simulink model "ASM_Traffic_new"  (R2024a)
settings: Solver=ode1  StartTime=SIM.tstart.v  StopTime=SIM.tend.v  FixedStep=SIM.StepSize.v  RelTol=1e-3
PostLoadFcn:
  | if any(exist('dsrtsu_mdlpostloadfcn', 'file') ~= 0), dsrtsu_mdlpostloadfcn('Execute', bdroot); end
  | try, asm_mdl_postloadfcn(bdroot, 'UpdateModel', 3600); catch, disp(lasterr); end,
InitFcn:
  | , if any(exist('rtifpga_mdlclblib', 'file') ~= 0), rtifpga_mdlclblib('Init', bdroot); end,
  | , if any(exist('dsmpb_private', 'file') ~= 0), dsmpb_private('dsmpb_mdlclblib', 'Init', bdroot); end,
undefined symbols (not defined in the file): _to_, a0b2, ASM_BrakeHydraulics_DemoSystems, ASM_VehicleDynamics_DemoSystems, b98103fe8ad365046cd0, BrakeCircuit, CPT, Crankshaft, DiscIntNeverNeededParam, dsmsi, FinalDriveAssembly, MDL, ModeSignals, Pos_BrakePedal_Maneuver, rad, RefSignals, s_to_rpm, SIM, SoftECU, Suspension, Tire, Transmission
libraries: ASM_Traffic_lib x135, simulink x100, ASM_Utils_lib x77, ASM_VehicleDynamics_lib x70, ASM_Environment_lib x22, dsmpblib x20, dsmsilib x15, MDLD_Utils_lib x10, ASM_BrakeHydraulics_lib x3
(part 49 of 63)

== system ASM_Traffic_new/Environment/Sensors/UserInterface/DISP_Plant/Object_Sensor_2D/Object_Sensor_2D_VisualizationData ==
  TrafficBus : Inport
  Bus Selector9 : BusSelector  OutputSignals=Object_Sensor_2D.Sensor_1_Front,Object_Sensor_2D.Sensor_2_Front_Left,Object_Sensor_2D.Sensor_3_Left,Object_Sensor_2D.Sensor_4_Rear_Left,Object_Sensor_2D.Sensor_5_Front_Right,Object_Sensor_2D.Sensor_6_Right,Object_Sensor_2D.Sensor_7_Rear_Right
  Sensor_1_Front_Long : Subsystem
  Sensor_2_Front_Left : Subsystem
  Sensor_3_Left : Subsystem
  Sensor_4_Rear_Left : Subsystem
  Sensor_5_Front_Right : Subsystem
  Sensor_6_Right : Subsystem
  Sensor_7_Rear_Right : Subsystem
  wires:
  Bus Selector9/1 -> Sensor_1_Front_Long/1(Sensor)  "<Sensor_1_Front>"
  TrafficBus/1 -> Bus Selector9/1
  Bus Selector9/2 -> Sensor_2_Front_Left/1(Sensor)  "<Sensor_2_Front_Left>"
  Bus Selector9/3 -> Sensor_3_Left/1(Sensor)  "<Sensor_3_Left>"
  Bus Selector9/4 -> Sensor_4_Rear_Left/1(Sensor)  "<Sensor_4_Rear_Left>"
  Bus Selector9/5 -> Sensor_5_Front_Right/1(Sensor)  "<Sensor_5_Front_Right>"
  Bus Selector9/6 -> Sensor_6_Right/1(Sensor)  "<Sensor_6_Right>"
  Bus Selector9/7 -> Sensor_7_Rear_Right/1(Sensor)  "<Sensor_7_Rear_Right>"

== system ASM_Traffic_new/Environment/Sensors/UserInterface/DISP_Plant/Object_Sensor_2D/Object_Type[] ==
  In1 : Inport
  Out1 : Outport  VectorParamsAs1DForOutWhenUnconnected=off
  wires:
  In1/1 -> Out1/1

== system ASM_Traffic_new/Environment/Sensors/UserInterface/DISP_Plant/Object_Sensor_2D/Object_Type[]1 ==
  In1 : Inport
  Out1 : Outport  VectorParamsAs1DForOutWhenUnconnected=off
  wires:
  In1/1 -> Out1/1

== system ASM_Traffic_new/Environment/Sensors/UserInterface/DISP_Plant/Object_Sensor_2D/Object_Type[]2 ==
  In1 : Inport
  Out1 : Outport  VectorParamsAs1DForOutWhenUnconnected=off
  wires:
  In1/1 -> Out1/1

== system ASM_Traffic_new/Environment/Sensors/UserInterface/DISP_Plant/Object_Sensor_2D/Object_Type[]3 ==
  In1 : Inport
  Out1 : Outport  VectorParamsAs1DForOutWhenUnconnected=off
  wires:
  In1/1 -> Out1/1

== system ASM_Traffic_new/Environment/Sensors/UserInterface/DISP_Plant/Object_Sensor_2D/Object_Type[]4 ==
  In1 : Inport
  Out1 : Outport  VectorParamsAs1DForOutWhenUnconnected=off
  wires:
  In1/1 -> Out1/1

== system ASM_Traffic_new/Environment/Sensors/UserInterface/DISP_Plant/Object_Sensor_2D/Object_Type[]5 ==
  In1 : Inport
  Out1 : Outport  VectorParamsAs1DForOutWhenUnconnected=off
  wires:
  In1/1 -> Out1/1

== system ASM_Traffic_new/Environment/Sensors/UserInterface/DISP_Plant/Object_Sensor_2D/Object_Type[]6 ==
  In1 : Inport
  Out1 : Outport  VectorParamsAs1DForOutWhenUnconnected=off
  wires:
  In1/1 -> Out1/1

== system ASM_Traffic_new/Environment/Sensors/UserInterface/DISP_Plant/Object_Sensor_2D/SensorEnable[0Off|1On] ==
  In1 : Inport
  Out1 : Outport  VectorParamsAs1DForOutWhenUnconnected=off
  wires:
  In1/1 -> Out1/1

== system ASM_Traffic_new/Environment/Sensors/UserInterface/DISP_Plant/Object_Sensor_2D/SensorIdx_Selected[] ==
  In1 : Inport
  Out1 : Outport  VectorParamsAs1DForOutWhenUnconnected=off
  wires:
  In1/1 -> Out1/1

== system ASM_Traffic_new/Environment/Sensors/UserInterface/DISP_Plant/Object_Sensor_2D/SensorSelection_Data[0|1] ==
  In1 : Inport
  Out1 : Outport  VectorParamsAs1DForOutWhenUnconnected=off
  wires:
  In1/1 -> Out1/1

== system ASM_Traffic_new/Environment/Sensors/UserInterface/DISP_Plant/Object_Sensor_2D/a_Rel[m|s2] ==
  In1 : Inport
  Out1 : Outport  VectorParamsAs1DForOutWhenUnconnected=off
  wires:
  In1/1 -> Out1/1

== system ASM_Traffic_new/Environment/Sensors/UserInterface/DISP_Plant/Object_Sensor_2D/a_Rel[m|s2]1 ==
  In1 : Inport
  Out1 : Outport  VectorParamsAs1DForOutWhenUnconnected=off
  wires:
  In1/1 -> Out1/1

== system ASM_Traffic_new/Environment/Sensors/UserInterface/DISP_Plant/Object_Sensor_2D/a_Rel[m|s2]2 ==
  In1 : Inport
  Out1 : Outport  VectorParamsAs1DForOutWhenUnconnected=off
  wires:
  In1/1 -> Out1/1

== system ASM_Traffic_new/Environment/Sensors/UserInterface/DISP_Plant/Object_Sensor_2D/a_Rel[m|s2]3 ==
  In1 : Inport
  Out1 : Outport  VectorParamsAs1DForOutWhenUnconnected=off
  wires:
  In1/1 -> Out1/1

== system ASM_Traffic_new/Environment/Sensors/UserInterface/DISP_Plant/Object_Sensor_2D/a_Rel[m|s2]4 ==
  In1 : Inport
  Out1 : Outport  VectorParamsAs1DForOutWhenUnconnected=off
  wires:
  In1/1 -> Out1/1

== system ASM_Traffic_new/Environment/Sensors/UserInterface/DISP_Plant/Object_Sensor_2D/a_Rel[m|s2]5 ==
  In1 : Inport
  Out1 : Outport  VectorParamsAs1DForOutWhenUnconnected=off
  wires:
  In1/1 -> Out1/1

== system ASM_Traffic_new/Environment/Sensors/UserInterface/DISP_Plant/Object_Sensor_2D/a_Rel[m|s2]6 ==
  In1 : Inport
  Out1 : Outport  VectorParamsAs1DForOutWhenUnconnected=off
  wires:
  In1/1 -> Out1/1

== system ASM_Traffic_new/Environment/Sensors/UserInterface/DISP_Plant/Object_Sensor_2D/v_Rel[m|s] ==
  In1 : Inport
  Out1 : Outport  VectorParamsAs1DForOutWhenUnconnected=off
  wires:
  In1/1 -> Out1/1

== system ASM_Traffic_new/Environment/Sensors/UserInterface/DISP_Plant/Object_Sensor_2D/v_Rel[m|s]1 ==
  In1 : Inport
  Out1 : Outport  VectorParamsAs1DForOutWhenUnconnected=off
  wires:
  In1/1 -> Out1/1

== system ASM_Traffic_new/Environment/Sensors/UserInterface/DISP_Plant/Object_Sensor_2D/v_Rel[m|s]2 ==
  In1 : Inport
  Out1 : Outport  VectorParamsAs1DForOutWhenUnconnected=off
  wires:
  In1/1 -> Out1/1

== system ASM_Traffic_new/Environment/Sensors/UserInterface/DISP_Plant/Object_Sensor_2D/v_Rel[m|s]3 ==
  In1 : Inport
  Out1 : Outport  VectorParamsAs1DForOutWhenUnconnected=off
  wires:
  In1/1 -> Out1/1

== system ASM_Traffic_new/Environment/Sensors/UserInterface/DISP_Plant/Object_Sensor_2D/v_Rel[m|s]4 ==
  In1 : Inport
  Out1 : Outport  VectorParamsAs1DForOutWhenUnconnected=off
  wires:
  In1/1 -> Out1/1

== system ASM_Traffic_new/Environment/Sensors/UserInterface/DISP_Plant/Object_Sensor_2D/v_Rel[m|s]5 ==
  In1 : Inport
  Out1 : Outport  VectorParamsAs1DForOutWhenUnconnected=off
  wires:
  In1/1 -> Out1/1

== system ASM_Traffic_new/Environment/Sensors/UserInterface/DISP_Plant/Object_Sensor_2D/v_Rel[m|s]6 ==
  In1 : Inport
  Out1 : Outport  VectorParamsAs1DForOutWhenUnconnected=off
  wires:
  In1/1 -> Out1/1

== system ASM_Traffic_new/Environment/Sensors/UserInterface/DISP_Plant/Object_Sensor_3D/Angle_Hor_Object[deg] ==
  In1 : Inport
  Out1 : Outport  VectorParamsAs1DForOutWhenUnconnected=off
  wires:
  In1/1 -> Out1/1

== system ASM_Traffic_new/Environment/Sensors/UserInterface/DISP_Plant/Object_Sensor_3D/Angle_Hor_Object[deg]1 ==
  In1 : Inport
  Out1 : Outport  VectorParamsAs1DForOutWhenUnconnected=off
  wires:
  In1/1 -> Out1/1

== system ASM_Traffic_new/Environment/Sensors/UserInterface/DISP_Plant/Object_Sensor_3D/Angle_Hor_Object[deg]2 ==
  In1 : Inport
  Out1 : Outport  VectorParamsAs1DForOutWhenUnconnected=off
  wires:
  In1/1 -> Out1/1

== system ASM_Traffic_new/Environment/Sensors/UserInterface/DISP_Plant/Object_Sensor_3D/Angle_Ver_Object[deg] ==
  In1 : Inport
  Out1 : Outport  VectorParamsAs1DForOutWhenUnconnected=off
  wires:
  In1/1 -> Out1/1

== system ASM_Traffic_new/Environment/Sensors/UserInterface/DISP_Plant/Object_Sensor_3D/Angle_Ver_Object[deg]1 ==
  In1 : Inport
  Out1 : Outport  VectorParamsAs1DForOutWhenUnconnected=off
  wires:
  In1/1 -> Out1/1

== system ASM_Traffic_new/Environment/Sensors/UserInterface/DISP_Plant/Object_Sensor_3D/Angle_Ver_Object[deg]2 ==
  In1 : Inport
  Out1 : Outport  VectorParamsAs1DForOutWhenUnconnected=off
  wires:
  In1/1 -> Out1/1

== system ASM_Traffic_new/Environment/Sensors/UserInterface/DISP_Plant/Object_Sensor_3D/Conflict_Flag[0|1] ==
  In1 : Inport
  Out1 : Outport  VectorParamsAs1DForOutWhenUnconnected=off
  wires:
  In1/1 -> Out1/1

== system ASM_Traffic_new/Environment/Sensors/UserInterface/DISP_Plant/Object_Sensor_3D/CycleConflict_Info[] ==
  In1 : Inport
  Out1 : Outport  VectorParamsAs1DForOutWhenUnconnected=off
  wires:
  In1/1 -> Out1/1

== system ASM_Traffic_new/Environment/Sensors/UserInterface/DISP_Plant/Object_Sensor_3D/DelayPulse_SensorOutput[0|1] ==
  In1 : Inport
  Out1 : Outport  VectorParamsAs1DForOutWhenUnconnected=off
  wires:
  In1/1 -> Out1/1

== system ASM_Traffic_new/Environment/Sensors/UserInterface/DISP_Plant/Object_Sensor_3D/Dist_Object[m] ==
  In1 : Inport
  Out1 : Outport  VectorParamsAs1DForOutWhenUnconnected=off
  wires:
  In1/1 -> Out1/1

== system ASM_Traffic_new/Environment/Sensors/UserInterface/DISP_Plant/Object_Sensor_3D/Dist_Object[m]1 ==
  In1 : Inport
  Out1 : Outport  VectorParamsAs1DForOutWhenUnconnected=off
  wires:
  In1/1 -> Out1/1

== system ASM_Traffic_new/Environment/Sensors/UserInterface/DISP_Plant/Object_Sensor_3D/Dist_Object[m]2 ==
  In1 : Inport
  Out1 : Outport  VectorParamsAs1DForOutWhenUnconnected=off
  wires:
  In1/1 -> Out1/1

== system ASM_Traffic_new/Environment/Sensors/UserInterface/DISP_Plant/Object_Sensor_3D/Flag_NearestPnt_Occluded[-1|0|1] ==
  In1 : Inport
  Out1 : Outport  VectorParamsAs1DForOutWhenUnconnected=off
  wires:
  In1/1 -> Out1/1

== system ASM_Traffic_new/Environment/Sensors/UserInterface/DISP_Plant/Object_Sensor_3D/Flag_NearestPnt_Occluded[-1|0|1]1 ==
  In1 : Inport
  Out1 : Outport  VectorParamsAs1DForOutWhenUnconnected=off
  wires:
  In1/1 -> Out1/1

== system ASM_Traffic_new/Environment/Sensors/UserInterface/DISP_Plant/Object_Sensor_3D/Flag_NearestPnt_Occluded[-1|0|1]2 ==
  In1 : Inport
  Out1 : Outport  VectorParamsAs1DForOutWhenUnconnected=off
  wires:
  In1/1 -> Out1/1

== system ASM_Traffic_new/Environment/Sensors/UserInterface/DISP_Plant/Object_Sensor_3D/Flag_Object_In_Scope[0Out|1In] ==
  In1 : Inport
  Out1 : Outport  VectorParamsAs1DForOutWhenUnconnected=off
  wires:
  In1/1 -> Out1/1

== system ASM_Traffic_new/Environment/Sensors/UserInterface/DISP_Plant/Object_Sensor_3D/Flag_Object_In_Scope[0Out|1In]1 ==
  In1 : Inport
  Out1 : Outport  VectorParamsAs1DForOutWhenUnconnected=off
  wires:
  In1/1 -> Out1/1

== system ASM_Traffic_new/Environment/Sensors/UserInterface/DISP_Plant/Object_Sensor_3D/Flag_Object_In_Scope[0Out|1In]2 ==
  In1 : Inport
  Out1 : Outport  VectorParamsAs1DForOutWhenUnconnected=off
  wires:
  In1/1 -> Out1/1

== system ASM_Traffic_new/Environment/Sensors/UserInterface/DISP_Plant/Object_Sensor_3D/Flag_Sensor_Apex_In_Object[0Out|1In] ==
  In1 : Inport
  Out1 : Outport  VectorParamsAs1DForOutWhenUnconnected=off
  wires:
  In1/1 -> Out1/1

== system ASM_Traffic_new/Environment/Sensors/UserInterface/DISP_Plant/Object_Sensor_3D/Flag_Sensor_Apex_In_Object[0Out|1In]1 ==
  In1 : Inport
  Out1 : Outport  VectorParamsAs1DForOutWhenUnconnected=off
  wires:
  In1/1 -> Out1/1

== system ASM_Traffic_new/Environment/Sensors/UserInterface/DISP_Plant/Object_Sensor_3D/Flag_Sensor_Apex_In_Object[0Out|1In]2 ==
  In1 : Inport
  Out1 : Outport  VectorParamsAs1DForOutWhenUnconnected=off
  wires:
  In1/1 -> Out1/1

== system ASM_Traffic_new/Environment/Sensors/UserInterface/DISP_Plant/Object_Sensor_3D/GetSensorData_3DSensor_1 ==
  TrafficBus : Inport
  Bus Selector1 : BusSelector  OutputSignals=Info.Flag_Object_In_Scope[0Out|1In],Info.Flag_Sensor_Apex_In_Object[0Out|1In],SensorOutput.Object_Info[-1None|1Fellow|2Static],SensorOutput.Object_ID[],SensorOutput.Object_Type[],SensorOutput.Dist_Object[m],SensorOutput.v_Rel_Object[m|s],SensorOutput.a_Rel_Object[m|s2],SensorOutput.Angle_Hor_Object[deg],SensorOutput.Angle_Ver_Object[deg],SensorOutput.Occlusion_Ratio_Object[-1|0_1],SensorOutput.Flag_NearestPnt_Occluded[-1|0|1]
  Flag_Object_In_Scope[0Out|1In] : Outport  VectorParamsAs1DForOutWhenUnconnected=off
  Flag_Sensor_Apex_In_Object[0Out|1In] : Outport  Port=2  VectorParamsAs1DForOutWhenUnconnected=off
  Object_Info[-1None|1Fellow|2Static] : Outport  Port=3  VectorParamsAs1DForOutWhenUnconnected=off
  Object_ID[] : Outport  Port=4  VectorParamsAs1DForOutWhenUnconnected=off
  Object_Type[] : Outport  Port=5  VectorParamsAs1DForOutWhenUnconnected=off
  Dist_Object[m] : Outport  Port=6  VectorParamsAs1DForOutWhenUnconnected=off
  v_Rel_Object[m|s] : Outport  Port=7  VectorParamsAs1DForOutWhenUnconnected=off
  a_Rel_Object[m|s2] : Outport  Port=8  VectorParamsAs1DForOutWhenUnconnected=off
  Angle_Hor_Object[deg] : Outport  Port=9  VectorParamsAs1DForOutWhenUnconnected=off
  Angle_Ver_Object[deg] : Outport  Port=10  VectorParamsAs1DForOutWhenUnconnected=off
  Occlusion_Ratio_Object[-1|0_1] : Outport  Port=11  VectorParamsAs1DForOutWhenUnconnected=off
  Flag_NearestPnt_Occluded[-1|0|1] : Outport  Port=12  VectorParamsAs1DForOutWhenUnconnected=off
  wires:
  Bus Selector1/12 -> Flag_NearestPnt_Occluded[-1|0|1]/1  "<Flag_NearestPnt_Occluded[-1|0|1]>"
  Bus Selector1/11 -> Occlusion_Ratio_Object[-1|0_1]/1  "<Occlusion_Ratio_Object[-1|0_1]>"
  TrafficBus/1 -> Bus Selector1/1
  Bus Selector1/1 -> Flag_Object_In_Scope[0Out|1In]/1  "<Flag_Object_In_Scope[0Out|1In]>"
  Bus Selector1/2 -> Flag_Sensor_Apex_In_Object[0Out|1In]/1  "<Flag_Sensor_Apex_In_Object[0Out|1In]>"
  Bus Selector1/3 -> Object_Info[-1None|1Fellow|2Static]/1  "<Object_Info[-1None|1Fellow|2Static]>"
  Bus Selector1/4 -> Object_ID[]/1  "<Object_ID[]>"
  Bus Selector1/5 -> Object_Type[]/1  "<Object_Type[]>"
  Bus Selector1/6 -> Dist_Object[m]/1  "<Dist_Object[m]>"
  Bus Selector1/7 -> v_Rel_Object[m|s]/1  "<v_Rel_Object[m|s]>"
  Bus Selector1/8 -> a_Rel_Object[m|s2]/1  "<a_Rel_Object[m|s2]>"
  Bus Selector1/9 -> Angle_Hor_Object[deg]/1  "<Angle_Hor_Object[deg]>"
  Bus Selector1/10 -> Angle_Ver_Object[deg]/1  "<Angle_Ver_Object[deg]>"

== system ASM_Traffic_new/Environment/Sensors/UserInterface/DISP_Plant/Object_Sensor_3D/GetSensorData_3DSensor_2 ==
  TrafficBus : Inport
  Bus Selector1 : BusSelector  OutputSignals=Info.Flag_Object_In_Scope[0Out|1In],Info.Flag_Sensor_Apex_In_Object[0Out|1In],SensorOutput.Object_Info[-1None|1Fellow|2Static],SensorOutput.Object_ID[],SensorOutput.Object_Type[],SensorOutput.Dist_Object[m],SensorOutput.v_Rel_Object[m|s],SensorOutput.a_Rel_Object[m|s2],SensorOutput.Angle_Hor_Object[deg],SensorOutput.Angle_Ver_Object[deg],SensorOutput.Occlusion_Ratio_Object[-1|0_1],SensorOutput.Flag_NearestPnt_Occluded[-1|0|1]
  Flag_Object_In_Scope[0Out|1In] : Outport  VectorParamsAs1DForOutWhenUnconnected=off
  Flag_Sensor_Apex_In_Object[0Out|1In] : Outport  Port=2  VectorParamsAs1DForOutWhenUnconnected=off
  Object_Info[-1None|1Fellow|2Static] : Outport  Port=3  VectorParamsAs1DForOutWhenUnconnected=off
  Object_ID[] : Outport  Port=4  VectorParamsAs1DForOutWhenUnconnected=off
  Object_Type[] : Outport  Port=5  VectorParamsAs1DForOutWhenUnconnected=off
  Dist_Object[m] : Outport  Port=6  VectorParamsAs1DForOutWhenUnconnected=off
  v_Rel_Object[m|s] : Outport  Port=7  VectorParamsAs1DForOutWhenUnconnected=off
  a_Rel_Object[m|s2] : Outport  Port=8  VectorParamsAs1DForOutWhenUnconnected=off
  Angle_Hor_Object[deg] : Outport  Port=9  VectorParamsAs1DForOutWhenUnconnected=off
  Angle_Ver_Object[deg] : Outport  Port=10  VectorParamsAs1DForOutWhenUnconnected=off
  Occlusion_Ratio_Object[-1|0_1] : Outport  Port=11  VectorParamsAs1DForOutWhenUnconnected=off
  Flag_NearestPnt_Occluded[-1|0|1] : Outport  Port=12  VectorParamsAs1DForOutWhenUnconnected=off
  wires:
  Bus Selector1/12 -> Flag_NearestPnt_Occluded[-1|0|1]/1  "<Flag_NearestPnt_Occluded[-1|0|1]>"
  Bus Selector1/11 -> Occlusion_Ratio_Object[-1|0_1]/1  "<Occlusion_Ratio_Object[-1|0_1]>"
  TrafficBus/1 -> Bus Selector1/1
  Bus Selector1/1 -> Flag_Object_In_Scope[0Out|1In]/1  "<Flag_Object_In_Scope[0Out|1In]>"
  Bus Selector1/2 -> Flag_Sensor_Apex_In_Object[0Out|1In]/1  "<Flag_Sensor_Apex_In_Object[0Out|1In]>"
  Bus Selector1/3 -> Object_Info[-1None|1Fellow|2Static]/1  "<Object_Info[-1None|1Fellow|2Static]>"
  Bus Selector1/4 -> Object_ID[]/1  "<Object_ID[]>"
  Bus Selector1/5 -> Object_Type[]/1  "<Object_Type[]>"
  Bus Selector1/6 -> Dist_Object[m]/1  "<Dist_Object[m]>"
  Bus Selector1/7 -> v_Rel_Object[m|s]/1  "<v_Rel_Object[m|s]>"
  Bus Selector1/8 -> a_Rel_Object[m|s2]/1  "<a_Rel_Object[m|s2]>"
  Bus Selector1/9 -> Angle_Hor_Object[deg]/1  "<Angle_Hor_Object[deg]>"
  Bus Selector1/10 -> Angle_Ver_Object[deg]/1  "<Angle_Ver_Object[deg]>"

== system ASM_Traffic_new/Environment/Sensors/UserInterface/DISP_Plant/Object_Sensor_3D/GetSensorData_3DSensor_3 ==
  TrafficBus : Inport
  Bus Selector1 : BusSelector  OutputSignals=Info.Flag_Object_In_Scope[0Out|1In],Info.Flag_Sensor_Apex_In_Object[0Out|1In],SensorOutput.Object_Info[-1None|1Fellow|2Static],SensorOutput.Object_ID[],SensorOutput.Object_Type[],SensorOutput.Dist_Object[m],SensorOutput.v_Rel_Object[m|s],SensorOutput.a_Rel_Object[m|s2],SensorOutput.Angle_Hor_Object[deg],SensorOutput.Angle_Ver_Object[deg],SensorOutput.Occlusion_Ratio_Object[-1|0_1],SensorOutput.Flag_NearestPnt_Occluded[-1|0|1]
  Flag_Object_In_Scope[0Out|1In] : Outport  VectorParamsAs1DForOutWhenUnconnected=off
  Flag_Sensor_Apex_In_Object[0Out|1In] : Outport  Port=2  VectorParamsAs1DForOutWhenUnconnected=off
  Object_Info[-1None|1Fellow|2Static] : Outport  Port=3  VectorParamsAs1DForOutWhenUnconnected=off
  Object_ID[] : Outport  Port=4  VectorParamsAs1DForOutWhenUnconnected=off
  Object_Type[] : Outport  Port=5  VectorParamsAs1DForOutWhenUnconnected=off
  Dist_Object[m] : Outport  Port=6  VectorParamsAs1DForOutWhenUnconnected=off
  v_Rel_Object[m|s] : Outport  Port=7  VectorParamsAs1DForOutWhenUnconnected=off
  a_Rel_Object[m|s2] : Outport  Port=8  VectorParamsAs1DForOutWhenUnconnected=off
  Angle_Hor_Object[deg] : Outport  Port=9  VectorParamsAs1DForOutWhenUnconnected=off
  Angle_Ver_Object[deg] : Outport  Port=10  VectorParamsAs1DForOutWhenUnconnected=off
  Occlusion_Ratio_Object[-1|0_1] : Outport  Port=11  VectorParamsAs1DForOutWhenUnconnected=off
  Flag_NearestPnt_Occluded[-1|0|1] : Outport  Port=12  VectorParamsAs1DForOutWhenUnconnected=off
  wires:
  Bus Selector1/12 -> Flag_NearestPnt_Occluded[-1|0|1]/1  "<Flag_NearestPnt_Occluded[-1|0|1]>"
  Bus Selector1/11 -> Occlusion_Ratio_Object[-1|0_1]/1  "<Occlusion_Ratio_Object[-1|0_1]>"
  TrafficBus/1 -> Bus Selector1/1
  Bus Selector1/1 -> Flag_Object_In_Scope[0Out|1In]/1  "<Flag_Object_In_Scope[0Out|1In]>"
  Bus Selector1/2 -> Flag_Sensor_Apex_In_Object[0Out|1In]/1  "<Flag_Sensor_Apex_In_Object[0Out|1In]>"
  Bus Selector1/3 -> Object_Info[-1None|1Fellow|2Static]/1  "<Object_Info[-1None|1Fellow|2Static]>"
  Bus Selector1/4 -> Object_ID[]/1  "<Object_ID[]>"
  Bus Selector1/5 -> Object_Type[]/1  "<Object_Type[]>"
  Bus Selector1/6 -> Dist_Object[m]/1  "<Dist_Object[m]>"
  Bus Selector1/7 -> v_Rel_Object[m|s]/1  "<v_Rel_Object[m|s]>"
  Bus Selector1/8 -> a_Rel_Object[m|s2]/1  "<a_Rel_Object[m|s2]>"
  Bus Selector1/9 -> Angle_Hor_Object[deg]/1  "<Angle_Hor_Object[deg]>"
  Bus Selector1/10 -> Angle_Ver_Object[deg]/1  "<Angle_Ver_Object[deg]>"
